simulink model "ASM_Traffic_MultiCore"  (R2026a)
settings: Solver=ode1  StartTime=SIM.tstart.v  StopTime=SIM.tend.v  FixedStep=SIM.StepSize.v
PostLoadFcn:
  | if any(exist('dsrtsu_mdlpostloadfcn', 'file') ~= 0), dsrtsu_mdlpostloadfcn('Execute', bdroot); end
  | try, asm_mdl_postloadfcn(bdroot, 'UpdateModel', 3600); catch, disp(lasterr); end,
InitFcn:
  | , if any(exist('rtifpga_mdlclblib', 'file') ~= 0), rtifpga_mdlclblib('Init', bdroot); end,
  | , if any(exist('dsmpb_private', 'file') ~= 0), dsmpb_private('dsmpb_mdlclblib', 'Init', bdroot); end,
model workspace (MAT data in the model file):
  asmReferencePath = [0 0.01 0.02 0.03 0.04 0.05 0.06 0.07 0.08 0.09 0.1 0.11 ... (350007 elements, 50001x7)]
  roadBounds : Simulink.Parameter (value not decoded)
  safetyAxes : Simulink.Parameter (value not decoded)
undefined symbols (not defined in the file): _to_, a0b2, ASM_BrakeHydraulics_DemoSystems, ASM_VehicleDynamics_DemoSystems, b98103fe8ad365046cd0, BrakeCircuit, controllerConfig, CPT, Crankshaft, DiscIntNeverNeededParam, dsmsi, FinalDriveAssembly, MDL, ModeSignals, mu, Pos_BrakePedal_Maneuver, rad, RefSignals, roadFamilyData, roadFamilyId, s_to_rpm, SIM, SoftECU, Suspension, Tire, Transmission
libraries: ASM_Traffic_lib x135, simulink x98, ASM_Utils_lib x77, ASM_VehicleDynamics_lib x70, ASM_Environment_lib x22, dsmpblib x20, dsmsilib x15, MDLD_Utils_lib x10, ASM_BrakeHydraulics_lib x3, sl_discontinuities x2
(part 33 of 65)

== system ASM_Traffic_MultiCore/VehicleDynamics/Plant/VehicleDynamics/Tire ==
  UnitVec_y_Wheel_CoorSys_V[FL,FR,RL,RR][x;y;z] : Inport
  RotationMatrix_V_to_E_T[3x3] : Inport  Port=2
  Pos_Wheels_CoorSys_E[FL,FR,RL,RR][x,y,z][m] : Inport  Port=3
  v_Abs_WheelBody_CoorSys_V[FL,FR,RL,RR][x;y;z][m|s] : Inport  Port=4
  w_Abs_Wheel_CoorSys_V[FL,FR,RL,RR][x,y,z][rad|s] : Inport  Port=5
  Sw_Tire_Parameter_Set[FL,FR,RL,RR][1|2|3|4] : Inport  Port=6
  Coef_Fric_Road[FL,FR,RL,RR][] : Inport  Port=7
  " Pos_z_CP_CoorSys_E[FL,FR,RL,RR][m]" : Inport  Port=8
  UnitVec_z_CP_CoorSys_E[FL,FR,RL,RR][x;y;z] : Inport  Port=9
  Reset[] : Inport  Port=10
  omega_Wheel[FL,FR,RL,RR][rad|s] : Inport  Port=11
  Sw_r_Tire[1:intern;2:extern] : Inport  Port=12
  r_Tire_extern[m] : Inport  Port=13
  ASMSignalCollector : Subsystem
  Bus Creator1 : BusCreator  Inputs=2
  Demux : Demux  Outputs=[1 1]
  Goto Tag Visibility : GotoTagVisibility  GotoTag=ASMBUS_VehicleDynamics_Tire_FL_ContactPoint
  Goto Tag Visibility1 : GotoTagVisibility  GotoTag=ASMBUS_VehicleDynamics_Tire_FL_Tire
  Goto Tag Visibility10 : GotoTagVisibility  GotoTag=ASMBUS_VehicleDynamics_Tire_RR_ForcesAndTorques
  Goto Tag Visibility16 : GotoTagVisibility  GotoTag=ASMBUS_VehicleDynamics_Tire_FR_ForcesAndTorques
  Goto Tag Visibility2 : GotoTagVisibility  GotoTag=ASMBUS_VehicleDynamics_Tire_FR_ContactPoint
  Goto Tag Visibility3 : GotoTagVisibility  GotoTag=ASMBUS_VehicleDynamics_Tire_FL_ForcesAndTorques
  Goto Tag Visibility4 : GotoTagVisibility  GotoTag=ASMBUS_VehicleDynamics_Tire_RL_ContactPoint
  Goto Tag Visibility5 : GotoTagVisibility  GotoTag=ASMBUS_VehicleDynamics_Tire_RL_Tire
  Goto Tag Visibility6 : GotoTagVisibility  GotoTag=ASMBUS_VehicleDynamics_Tire_FR_Tire
  Goto Tag Visibility7 : GotoTagVisibility  GotoTag=ASMBUS_VehicleDynamics_Tire_RL_ForcesAndTorques
  Goto Tag Visibility8 : GotoTagVisibility  GotoTag=ASMBUS_VehicleDynamics_Tire_RR_ContactPoint
  Goto Tag Visibility9 : GotoTagVisibility  GotoTag=ASMBUS_VehicleDynamics_Tire_RR_Tire
  Mux{1,3..5} (4 alike) : Mux
  Sat_TireParSet : Saturate  UpperLimit=4  LowerLimit=1
  Selector{1..2,14,32} (4 alike) : Selector  InputPortWidth=4  IndexOptions=Index vector (dialog)  Indices=[2]  OutputSizes=1
  Selector{3,9..10,31} (4 alike) : Selector  InputPortWidth=4  IndexOptions=Index vector (dialog)  Indices=[1]  OutputSizes=1
  Selector{7..8,11..13} (5 alike) : Selector  InputPortWidth=12  IndexOptions=Index vector (dialog)  Indices=[4 5 6]  OutputSizes=1
  Selector{15..16,22,33} (4 alike) : Selector  InputPortWidth=4  IndexOptions=Index vector (dialog)  Indices=[3]  OutputSizes=1
  Selector{17..21} (5 alike) : Selector  InputPortWidth=12  IndexOptions=Index vector (dialog)  Indices=[7 8 9]  OutputSizes=1
  Selector{23..25,34} (4 alike) : Selector  InputPortWidth=4  IndexOptions=Index vector (dialog)  Indices=[4]  OutputSizes=1
  Selector{26..30} (5 alike) : Selector  InputPortWidth=12  IndexOptions=Index vector (dialog)  Indices=[10 11 12]  OutputSizes=1
  Selector{4..6,37..38} (5 alike) : Selector  InputPortWidth=12  IndexOptions=Index vector (dialog)  Indices=[1 2 3]  OutputSizes=1
  TIRE_MODE : ASM_VehicleDynamics_lib/VehicleDynamics/Tire/Base/TIRE_MODE  Tag=ASM_SUBCOMPONENT  ModeLeft=MDL.VehicleDynamics.Tire.ModeLeft  ModeRight=MDL.VehicleDynamics.Tire.ModeRight  ASMProperties=struct('Name','TIRE_MODE','Version','1.0','Library','ASM_VehicleDynamics_lib')  ASMInstanceName=tire_mode  ASMInstanceID=1
  Tire_FL : Subsystem
  Tire_FR : Subsystem
  Tire_RL : Subsystem
  Tire_RR : Subsystem
  p[Pa] : Constant  Value=220000
  ASMSignalBus : Outport  VectorParamsAs1DForOutWhenUnconnected=off
  F_Tire_CoorSys_V[FL,FR,RL,RR][x;y;z][N] : Outport  Port=2  VectorParamsAs1DForOutWhenUnconnected=off
  Trq_Tire_CoorSys_V[FL,FR,RL,RR][x;y;z][Nm] : Outport  Port=3  VectorParamsAs1DForOutWhenUnconnected=off
  Stiffness_z_Tire[FL,FR,RL,RR][N|m] : Outport  Port=4  VectorParamsAs1DForOutWhenUnconnected=off
  Trq_Tire_Wheel[FL,FR,RL,RR][Nm] : Outport  Port=5  VectorParamsAs1DForOutWhenUnconnected=off
  wires:
  ASMSignalCollector/1(ASMSignalBus) -> ASMSignalBus/1
  Mux4/1 -> F_Tire_CoorSys_V[FL,FR,RL,RR][x;y;z][N]/1
  Mux1/1 -> Trq_Tire_CoorSys_V[FL,FR,RL,RR][x;y;z][Nm]/1
  Selector10/1 -> Tire_FL/9(omega_Wheel[rad|s])
  omega_Wheel[FL,FR,RL,RR][rad|s]/1 -> Selector24/1, Selector22/1, Selector1/1, Selector10/1
  Selector37/1 -> Tire_FL/8(UnitVec_y_Wheel_CoorSys_V[x;y;z])
  UnitVec_y_Wheel_CoorSys_V[FL,FR,RL,RR][x;y;z]/1 -> Selector30/1, Selector21/1, Selector7/1, Selector37/1
  RotationMatrix_V_to_E_T[3x3]/1 -> Tire_RR/7(RotationMatrix_V_to_E_T[3x3]), Tire_RL/7(RotationMatrix_V_to_E_T[3x3]), Tire_FR/7(RotationMatrix_V_to_E_T[3x3]), Tire_FL/7(RotationMatrix_V_to_E_T[3x3])
  UnitVec_z_CP_CoorSys_E[FL,FR,RL,RR][x;y;z]/1 -> Selector26/1, Selector17/1, Selector11/1, Selector4/1
  " Pos_z_CP_CoorSys_E[FL,FR,RL,RR][m]"/1 -> Selector25/1, Selector16/1, Selector2/1, Selector3/1
  Selector3/1 -> Tire_FL/2(" Pos_z_CP_CoorSys_E[m]")
  Selector9/1 -> Tire_FL/1(Coeff_Fric_Road[])
  Coef_Fric_Road[FL,FR,RL,RR][]/1 -> Selector23/1, Selector15/1, Selector14/1, Selector9/1
  Selector4/1 -> Tire_FL/3(UnitVec_z_CP_CoorSys_E[x;y;z])
  Pos_Wheels_CoorSys_E[FL,FR,RL,RR][x,y,z][m]/1 -> Selector27/1, Selector18/1, Selector12/1, Selector5/1
  Selector5/1 -> Tire_FL/4(Pos_Wheels_CoorSys_E[x;y;z][m])
  v_Abs_WheelBody_CoorSys_V[FL,FR,RL,RR][x;y;z][m|s]/1 -> Selector28/1, Selector19/1, Selector8/1, Selector6/1
  Selector6/1 -> Tire_FL/5(v_Abs_WheelBody_CoorSys_V[x;y;z][m|s])
  w_Abs_Wheel_CoorSys_V[FL,FR,RL,RR][x,y,z][rad|s]/1 -> Selector29/1, Selector20/1, Selector13/1, Selector38/1
  Selector38/1 -> Tire_FL/6(w_Abs_Wheel_CoorSys_V[x;y;z][rad|s])
  Selector14/1 -> Tire_FR/1(Coeff_Fric_Road[])
  Selector2/1 -> Tire_FR/2(" Pos_z_CP_CoorSys_E[m]")
  Selector11/1 -> Tire_FR/3(UnitVec_z_CP_CoorSys_E[x;y;z])
  Selector12/1 -> Tire_FR/4(Pos_Wheels_CoorSys_E[x;y;z][m])
  Selector8/1 -> Tire_FR/5(v_Abs_WheelBody_CoorSys_V[x;y;z][m|s])
  Selector13/1 -> Tire_FR/6(w_Abs_Wheel_CoorSys_V[x;y;z][rad|s])
  Selector7/1 -> Tire_FR/8(UnitVec_y_Wheel_CoorSys_V[x;y;z])
  Selector1/1 -> Tire_FR/9(omega_Wheel[rad|s])
  Selector15/1 -> Tire_RL/1(Coeff_Fric_Road[])
  Selector16/1 -> Tire_RL/2(" Pos_z_CP_CoorSys_E[m]")
  Selector17/1 -> Tire_RL/3(UnitVec_z_CP_CoorSys_E[x;y;z])
  Selector18/1 -> Tire_RL/4(Pos_Wheels_CoorSys_E[x;y;z][m])
  Selector19/1 -> Tire_RL/5(v_Abs_WheelBody_CoorSys_V[x;y;z][m|s])
  Selector20/1 -> Tire_RL/6(w_Abs_Wheel_CoorSys_V[x;y;z][rad|s])
  Selector21/1 -> Tire_RL/8(UnitVec_y_Wheel_CoorSys_V[x;y;z])
  Selector22/1 -> Tire_RL/9(omega_Wheel[rad|s])
  Tire_FL/1(F_Tire[x;y;z][N]) -> Mux4/1
  Tire_FR/1(F_Tire[x;y;z][N]) -> Mux4/2
  Tire_RL/1(F_Tire[x;y;z][N]) -> Mux4/3
  Tire_RR/1(F_Tire[x;y;z][N]) -> Mux4/4
  Tire_FL/2(Trq_Tire[x;y;z][Nm]) -> Mux1/1
  Tire_FR/2(Trq_Tire[x;y;z][Nm]) -> Mux1/2
  Tire_RL/2(Trq_Tire[x;y;z][Nm]) -> Mux1/3
  Tire_RR/2(Trq_Tire[x;y;z][Nm]) -> Mux1/4
  Mux3/1 -> Trq_Tire_Wheel[FL,FR,RL,RR][Nm]/1
  Tire_FL/3(Trq_Tire_Wheel[Nm]) -> Mux3/1
  Tire_FR/3(Trq_Tire_Wheel[Nm]) -> Mux3/2
  Tire_RL/3(Trq_Tire_Wheel[Nm]) -> Mux3/3
  Tire_RR/3(Trq_Tire_Wheel[Nm]) -> Mux3/4
  Sw_Tire_Parameter_Set[FL,FR,RL,RR][1|2|3|4]/1 -> Sat_TireParSet/1
  Selector31/1 -> Tire_FL/10(Sw_Tire_Parameter_Set[1|2|3|4])
  Selector32/1 -> Tire_FR/10(Sw_Tire_Parameter_Set[1|2|3|4])
  Selector33/1 -> Tire_RL/10(Sw_Tire_Parameter_Set[1|2|3|4])
  Selector34/1 -> Tire_RR/10(Sw_Tire_Parameter_Set[1|2|3|4])
  Selector30/1 -> Tire_RR/8(UnitVec_y_Wheel_CoorSys_V[x;y;z])
  Selector24/1 -> Tire_RR/9(omega_Wheel[rad|s])
  Selector29/1 -> Tire_RR/6(w_Abs_Wheel_CoorSys_V[x;y;z][rad|s])
  Selector28/1 -> Tire_RR/5(v_Abs_WheelBody_CoorSys_V[x;y;z][m|s])
  Selector27/1 -> Tire_RR/4(Pos_Wheels_CoorSys_E[x;y;z][m])
  Selector26/1 -> Tire_RR/3(UnitVec_z_CP_CoorSys_E[x;y;z])
  Selector25/1 -> Tire_RR/2(" Pos_z_CP_CoorSys_E[m]")
  Selector23/1 -> Tire_RR/1(Coeff_Fric_Road[])
  Tire_FL/4(Stiffness_z_Tire[N|m]) -> Mux5/1
  Tire_FR/4(Stiffness_z_Tire[N|m]) -> Mux5/2
  Tire_RL/4(Stiffness_z_Tire[N|m]) -> Mux5/3
  Tire_RR/4(Stiffness_z_Tire[N|m]) -> Mux5/4
  Mux5/1 -> Stiffness_z_Tire[FL,FR,RL,RR][N|m]/1
  Reset[]/1 -> Tire_RR/11(Reset[]), Tire_RL/11(Reset[]), Tire_FR/11(Reset[]), Tire_FL/11(Reset[])
  Sat_TireParSet/1 -> Selector34/1, Selector33/1, Selector32/1, Selector31/1
  Demux/1 -> Tire_RL/12(Mode[1Normal|2Mirror|3Symmetric]), Tire_FL/12(Mode[1Normal|2Mirror|3Symmetric])
  p[Pa]/1 -> Tire_RR/13(p[Pa]), Tire_RL/13(p[Pa]), Tire_FR/13(p[Pa]), Tire_FL/13(p[Pa])
  Demux/2 -> Tire_RR/12(Mode[1Normal|2Mirror|3Symmetric]), Tire_FR/12(Mode[1Normal|2Mirror|3Symmetric])
  TIRE_MODE/1 -> Demux/1
  Sw_r_Tire[1:intern;2:extern]/1 -> Bus Creator1/1
  r_Tire_extern[m]/1 -> Bus Creator1/2
  Bus Creator1/1 -> Tire_RR/14(Tire_Switches), Tire_RL/14(Tire_Switches), Tire_FR/14(Tire_Switches), Tire_FL/14(Tire_Switches)

== system ASM_Traffic_MultiCore/VehicleDynamics/Plant/VehicleDynamics/TireMapping_CP ==
  Sw_Tire_Parameter_Set_CP[:][1|2|3|4] : Inport
  Fric_Coeff_CP[:][] : Inport  Port=2
  Pos_z_CP[:][m] : Inport  Port=3
  UnitVec_z_CP[:][x;y;z] : Inport  Port=4
  Selector : Selector  IndexOptions=Index vector (dialog)  Indices=[1:4]  OutputSizes=1
  Selector1 : Selector  IndexOptions=Index vector (dialog)  Indices=[1:4]  OutputSizes=1
  Selector2 : Selector  IndexOptions=Index vector (dialog)  Indices=[1:4]  OutputSizes=1
  Selector3 : Selector  IndexOptions=Index vector (dialog)  Indices=[1:12]  OutputSizes=1
  Sw_Tire_Parameter_Set_CP_Veh[FL;FR;RL;RR][1|2|3|4] : Outport  VectorParamsAs1DForOutWhenUnconnected=off
  Fric_Coeff_CP_Veh[FL;FR;RL;RR][] : Outport  Port=2  VectorParamsAs1DForOutWhenUnconnected=off
  Pos_z_CP_Veh[FL;FR;RL;RR][m] : Outport  Port=3  VectorParamsAs1DForOutWhenUnconnected=off
  UnitVec_z_CP_Veh[FL;FR;RL;RR][x;y;z] : Outport  Port=4  VectorParamsAs1DForOutWhenUnconnected=off
  wires:
  Selector2/1 -> Sw_Tire_Parameter_Set_CP_Veh[FL;FR;RL;RR][1|2|3|4]/1
  Selector3/1 -> UnitVec_z_CP_Veh[FL;FR;RL;RR][x;y;z]/1
  Selector1/1 -> Fric_Coeff_CP_Veh[FL;FR;RL;RR][]/1
  Selector/1 -> Pos_z_CP_Veh[FL;FR;RL;RR][m]/1
  Pos_z_CP[:][m]/1 -> Selector/1
  Fric_Coeff_CP[:][]/1 -> Selector1/1
  UnitVec_z_CP[:][x;y;z]/1 -> Selector3/1
  Sw_Tire_Parameter_Set_CP[:][1|2|3|4]/1 -> Selector2/1

== system ASM_Traffic_MultiCore/VehicleDynamics/Plant/VehicleDynamics/VehicleInits ==
  q_dt_Vehicle_Init[6x1] : Inport
  q_dt_Wheel_Init[:] : Inport  Port=2
  q_Wheel_Init_In[:] : Inport  Port=3
  Bus Selector : BusSelector  OutputSignals=Tire_allSignals.Tire_FL.Tire.r_Dyn_Tire[m],Tire_allSignals.Tire_FR.Tire.r_Dyn_Tire[m],Tire_allSignals.Tire_RL.Tire.r_Dyn_Tire[m],Tire_allSignals.Tire_RR.Tire.r_Dyn_Tire[m]
  Mux : Mux  Inputs=2
  Mux1 : Mux
  Product : Product  Inputs=/*  RndMeth=Zero
  Saturation : Saturate  UpperLimit=inf  LowerLimit=0.01
  Unit Delay : UnitDelay  SampleTime=-1
  v_x_Init[m|s] : Selector  InputPortWidth=6  IndexOptions=Index vector (dialog)  Indices=[1]  OutputSizes=1
  omega_Wheel_Init[:][rad|s] : Outport  VectorParamsAs1DForOutWhenUnconnected=off
  q_dt_Init[:] : Outport  Port=2  VectorParamsAs1DForOutWhenUnconnected=off
  q_Wheel_Init[:] : Outport  Port=3  VectorParamsAs1DForOutWhenUnconnected=off
  wires:
  q_dt_Vehicle_Init[6x1]/1 -> v_x_Init[m|s]/1, Mux/1
  Mux1/1 -> Saturation/1
  Bus Selector/4 -> Mux1/4  "<r_Dyn_Tire[m]>"
  Bus Selector/3 -> Mux1/3  "<r_Dyn_Tire[m]>"
  Bus Selector/2 -> Mux1/2  "<r_Dyn_Tire[m]>"
  v_x_Init[m|s]/1 -> Product/2
  Mux/1 -> q_dt_Init[:]/1
  q_Wheel_Init_In[:]/1 -> q_Wheel_Init[:]/1
  q_dt_Wheel_Init[:]/1 -> Mux/2
  Saturation/1 -> Product/1
  Bus Selector/1 -> Mux1/1  "<r_Dyn_Tire[m]>"
  Unit Delay/1 -> omega_Wheel_Init[:][rad|s]/1
  Product/1 -> Unit Delay/1
  [ASMBUS_VehicleDynamics_Tire] -> Bus Selector/1

== system ASM_Traffic_MultiCore/VehicleDynamics/Plant/VehicleDynamics/VehicleMovement ==
  F_Aero_CoorSys_V[x;y;z][N] : Inport
  Trq_Aero_CoorSys_V[x;y;z][Nm] : Inport  Port=2
  F_Tire_CoorSys_V[FL,FR,RL,RR][x;y;z][N] : Inport  Port=3
  Trq_Tire_CoorSys_V[FL,FR,RL,RR][x;y;z][Nm] : Inport  Port=4
  Stiffness_z_Tire[FL,FR,RL,RR][N|m] : Inport  Port=5
  w_Wheel[FL,FR,RL,RR][x;y;z][rad|s] : Inport  Port=6
  Trq_Shaft_CoorSys_V[FL,FR,RL,RR][x;y;z][Nm] : Inport  Port=7
  gF_Susp[q1_Front;q2_Front;q1_Rear;q2_Rear][] : Inport  Port=8
  Pos_Wheel[FL,FR,RL,RR][x;y;z][m] : Inport  Port=9
  w_Rel_WheelBody[FL,FR,RL,RR][x y z][rad|s] : Inport  Port=10
  v_Rel_WheelBody[FL,FR,RL,RR][x;y;z][m|s] : Inport  Port=11
  Pos_Vehicle_Init_CoorSys_E[x;y;z][m] : Inport  Port=12
  Angle_V_Init_CoorSys_E[x;y;z][rad] : Inport  Port=13
  Reset[] : Inport  Port=14
  KeepVehiclePosition[0|1] : Inport  Port=15
  gRear_dq_Rear_dt[2x2][] : Inport  Port=16
  gFront_dq_Front_dt[2x2][] : Inport  Port=17
  SuspensionKinematicsRelations_Rear : Inport  Port=18
  SuspensionKinematicsRelations_Front : Inport  Port=19
  F_External_CoorSys_V[x,y,z][N] : Inport  Port=20
  Trq_External_CoorSys_V[x,y,z][Nm] : Inport  Port=21
  Stabilization_F_External[3X6] : Inport  Port=22
  Stabilization_Trq_External[3X6] : Inport  Port=23
  q_dt_Init[:] : Inport  Port=24
  q_Wheel_Init[:] : Inport  Port=25
  ASMSignalCollector : Subsystem
  Bus Selector1 : BusSelector  OutputSignals=Pos_RL_Wheel_dq_Rear[q1;q2][x;y;z][],w_Rel_RL_Wheel_dq_Rear_dt[q1;q2][x;y;z][],Pos_RR_Wheel_dq_Rear[q1;q2][x;y;z][],w_Rel_RR_Wheel_dq_Rear[q1;q2][x;y;z][]
  Bus Selector2 : BusSelector  OutputSignals=Pos_FL_Wheel_dq_Front[q1;q2][x;y;z][],w_Rel_FL_Wheel_dq_Front_dt[q1;q2][x;y;z][],Pos_FR_Wheel_dq_Front[q1;q2][x;y;z][],w_Rel_FR_Wheel_dq_Front[q1;q2][x;y;z][]
  COORDINATE_TRANSFORMATION : ASM_VehicleDynamics_lib/VehicleDynamics/VehicleMovement/COORDINATE_TRANSFORMATION  Tag=ASM_SUBCOMPONENT  StepSize=SIM.StepSize  ASMProperties=struct('Name','COORDINATE_TRANSFORMATION','Version','5.0','Library','ASM_VehicleDynamics_lib')  ASMInstanceName=coordinate_transformation  ASMInstanceID=1
  Goto Tag Visibility : GotoTagVisibility  GotoTag=ASMBUS_VehicleDynamics_VehicleMotion
  Goto Tag Visibility1 : GotoTagVisibility  GotoTag=ASMBUS_VehicleDynamics_CoGAndWheelVelocities
  Goto Tag Visibility2 : GotoTagVisibility  GotoTag=ASMBUS_VehicleDynamics_SensorMotion
  Goto Tag Visibility3 : GotoTagVisibility  GotoTag=ASMBUS_VehicleDynamics_MassForcesAndTorques
  Goto Tag Visibility4 : GotoTagVisibility  GotoTag=ASMBUS_VehicleDynamics_CoordinateTransformation
  Goto Tag Visibility5 : GotoTagVisibility  GotoTag=ASMBUS_VehicleDynamics_VehicleMass
  J : Constant  Value=zeros(3,3)
  MASS_FORCES_AND_TORQUES : ASM_VehicleDynamics_lib/VehicleDynamics/VehicleMovement/MASS_FORCES_AND_TORQUES  Tag=ASM_SUBCOMPONENT  ASMProperties=struct('Name','MASS_FORCES_AND_TORQUES','Version','3.0','Library','ASM_VehicleDynamics_lib')  ASMInstanceName=mass_forces_and_torques  ASMInstanceID=1
  OR : Subsystem
  SENSOR_MOTION : ASM_VehicleDynamics_lib/VehicleDynamics/VehicleMovement/SENSOR_MOTION  Tag=ASM_SUBCOMPONENT  Const_PosVec_Sensor1=MDL.VehicleDynamics.VehicleMovement.SensorMotion.Const_PosVec_Sensor1  Const_PosVec_Sensor2=MDL.VehicleDynamics.VehicleMovement.SensorMotion.Const_PosVec_Sensor2  Const_PosVec_Sensor3=MDL.VehicleDynamics.VehicleMovement.SensorMotion.Const_PosVec_Sensor3  Const_PosVec_Sensor4=MDL.VehicleDynamics.VehicleMovement.SensorMotion.Const_PosVec_Sensor4  ASMProperties=struct('Name','SENSOR_MOTION','Version','5.0','Library','ASM_VehicleDynamics_lib')  ASMInstanceName=sensor_motion  ASMInstanceID=1
  Selector1 : Selector  InputPortWidth=15  IndexOptions=Index vector (dialog)  Indices=[4:15]  OutputSizes=1
  Selector2 : Selector  InputPortWidth=15  IndexOptions=Index vector (dialog)  Indices=[4:15]  OutputSizes=1
  Selector3 : Selector  InputPortWidth=15  IndexOptions=Index vector (dialog)  Indices=[4:15]  OutputSizes=1
  Sw_TestBenchMode[1Vehicle|2TestBench] : Constant
  Terminator : Terminator
  VEHICLE_AND_WHEEL_VELOCITIES : ASM_VehicleDynamics_lib/VehicleDynamics/VehicleMovement/VEHICLE_AND_WHEEL_VELOCITIES  Tag=ASM_SUBCOMPONENT  ASMProperties=struct('Name','VEHICLE_AND_WHEEL_VELOCITIES','Version','1.0','Library','ASM_VehicleDynamics_lib')  ASMInstanceName=vehicle_and_wheel_velocities  ASMInstanceID=1
  VEHICLE_MASS_AND_ADDITIONAL_LOADS : ASM_VehicleDynamics_lib/VehicleDynamics/VehicleMovement/VEHICLE_MASS_AND_ADDITIONAL_LOADS  Tag=ASM_SUBCOMPONENT  Const_m_Vehicle=MDL.VehicleDynamics.Vehicle.Const_m_Vehicle  Const_PosVec_CoG_Vehicle=MDL.VehicleDynamics.Vehicle.Const_PosVec_CoG_Vehicle  Const_Inertia_Tensor_Vehicle=MDL.VehicleDynamics.Vehicle.Const_Inertia_Tensor_Vehicle  Const_m_AddLoad1=MDL.VehicleDynamics.VehicleMovement.AddLoad1.Const_m_AddLoad1  Const_PosVec_CoG_AddLoad1=MDL.VehicleDynamics.VehicleMovement.AddLoad1.Const_PosVec_CoG_AddLoad1  Const_Inertia_Tensor_AddLoad1=MDL.VehicleDynamics.VehicleMovement.AddLoad1.Const_Inertia_Tensor_AddLoad1  Sw_AddLoad1=MDL.VehicleDynamics.VehicleMovement.AddLoad1.Sw_AddLoad1  Const_m_AddLoad2=MDL.VehicleDynamics.VehicleMovement.AddLoad2.Const_m_AddLoad2  Const_PosVec_CoG_AddLoad2=MDL.VehicleDynamics.VehicleMovement.AddLoad2.Const_PosVec_CoG_AddLoad2  Const_Inertia_Tensor_AddLoad2=MDL.VehicleDynamics.VehicleMovement.AddLoad2.Const_Inertia_Tensor_AddLoad2  Sw_AddLoad2=MDL.VehicleDynamics.VehicleMovement.AddLoad2.Sw_AddLoad2  Const_m_AddLoad3=MDL.VehicleDynamics.VehicleMovement.AddLoad3.Const_m_AddLoad3  Const_PosVec_CoG_AddLoad3=MDL.VehicleDynamics.VehicleMovement.AddLoad3.Const_PosVec_CoG_AddLoad3  Const_Inertia_Tensor_AddLoad3=MDL.VehicleDynamics.VehicleMovement.AddLoad3.Const_Inertia_Tensor_AddLoad3  Sw_AddLoad3=MDL.VehicleDynamics.VehicleMovement.AddLoad3.Sw_AddLoad3  Const_m_AddLoad4=MDL.VehicleDynamics.VehicleMovement.AddLoad4.Const_m_AddLoad4  Const_PosVec_CoG_AddLoad4=MDL.VehicleDynamics.VehicleMovement.AddLoad4.Const_PosVec_CoG_AddLoad4  Const_Inertia_Tensor_AddLoad4=MDL.VehicleDynamics.VehicleMovement.AddLoad4.Const_Inertia_Tensor_AddLoad4  Sw_AddLoad4=MDL.VehicleDynamics.VehicleMovement.AddLoad4.Sw_AddLoad4  Const_m_AddLoad5=MDL.VehicleDynamics.VehicleMovement.AddLoad5.Const_m_AddLoad5  Const_PosVec_CoG_AddLoad5=MDL.VehicleDynamics.VehicleMovement.AddLoad5.Const_PosVec_CoG_AddLoad5  Const_Inertia_Tensor_AddLoad5=MDL.VehicleDynamics.VehicleMovement.AddLoad5.Const_Inertia_Tensor_AddLoad5  Sw_AddLoad5=MDL.VehicleDynamics.VehicleMovement.AddLoad5.Sw_AddLoad5  Const_m_AddLoad6=MDL.VehicleDynamics.VehicleMovement.AddLoad6.Const_m_AddLoad6  Const_PosVec_CoG_AddLoad6=MDL.VehicleDynamics.VehicleMovement.AddLoad6.Const_PosVec_CoG_AddLoad6  Const_Inertia_Tensor_AddLoad6=MDL.VehicleDynamics.VehicleMovement.AddLoad6.Const_Inertia_Tensor_AddLoad6  Sw_AddLoad6=MDL.VehicleDynamics.VehicleMovement.AddLoad6.Sw_AddLoad6  ASMProperties=struct('Name','VEHICLE_MASS_AND_ADDITIONAL_LOADS','Version','4.0','Library','ASM_VehicleDynamics_lib')  ASMInstanceName=vehicle_mass_and_additional_loads  ASMInstanceID=1
  VEHICLE_MOTION_CAR : ASM_VehicleDynamics_lib/VehicleDynamics/VehicleMovement/VEHICLE_MOTION_CAR  Tag=ASM_SUBCOMPONENT  StepSize=SIM.StepSize  ASMProperties=struct('Name','VEHICLE_MOTION_CAR','Version','6.0','Library','ASM_VehicleDynamics_lib')  ASMInstanceName=vehicle_motion_car  ASMInstanceID=1
  m : Constant  Value=0
  r_CoG : Constant  Value=[0 0 0]
  ASMSignalBus : Outport  VectorParamsAs1DForOutWhenUnconnected=off
  v_Abs_Vehicle_CoG[x;y;z][m|s] : Outport  Port=2  VectorParamsAs1DForOutWhenUnconnected=off
  RotationMatrix_V_to_E_T[3x3] : Outport  Port=3  VectorParamsAs1DForOutWhenUnconnected=off
  Pos_Wheels_CoorSys_E[FL,FR,RL,RR][x;y;z][m] : Outport  Port=4  VectorParamsAs1DForOutWhenUnconnected=off
  v_Abs_WheelBody_CoorSys_V[FL,FR,RL,RR][x y z][m|s] : Outport  Port=5  VectorParamsAs1DForOutWhenUnconnected=off
  w_Abs_Wheel_CoorSys_V[FL,FR,RL,RR][x,y,z][rad|s] : Outport  Port=6  VectorParamsAs1DForOutWhenUnconnected=off
  F_Gyroscopic[FL,FR,RL,RR][x;y;z][N] : Outport  Port=7  VectorParamsAs1DForOutWhenUnconnected=off
  Trq_Gyroscopic[FL,FR,RL,RR][x;y;z][Nm] : Outport  Port=8  VectorParamsAs1DForOutWhenUnconnected=off
  F_Gravitational[FL,FR,RL,RR][x;y;z][N] : Outport  Port=9  VectorParamsAs1DForOutWhenUnconnected=off
  q_Wheel_dt[q1_Front;q2_Front;q1_Rear;q2_Rear][] : Outport  Port=10  VectorParamsAs1DForOutWhenUnconnected=off
  q_Wheel[q1_Front;q2_Front;q1_Rear;q2_Rear][] : Outport  Port=11  VectorParamsAs1DForOutWhenUnconnected=off
  tag scope: ASMBUS_VehicleDynamics_CoGAndWheelVelocities=scoped, ASMBUS_VehicleDynamics_CoordinateTransformation=scoped, ASMBUS_VehicleDynamics_MassForcesAndTorques=scoped, ASMBUS_VehicleDynamics_SensorMotion=scoped, ASMBUS_VehicleDynamics_VehicleMass=global, ASMBUS_VehicleDynamics_VehicleMotion=scoped
  wires:
  COORDINATE_TRANSFORMATION/1 -> [ASMBUS_VehicleDynamics_CoordinateTransformation]
  VEHICLE_AND_WHEEL_VELOCITIES/1 -> [ASMBUS_VehicleDynamics_CoGAndWheelVelocities]
  VEHICLE_MOTION_CAR/1 -> [ASMBUS_VehicleDynamics_VehicleMotion]
  VEHICLE_AND_WHEEL_VELOCITIES/3 -> w_Abs_Wheel_CoorSys_V[FL,FR,RL,RR][x,y,z][rad|s]/1
  VEHICLE_AND_WHEEL_VELOCITIES/5 -> MASS_FORCES_AND_TORQUES/2, v_Abs_Vehicle_CoG[x;y;z][m|s]/1
  VEHICLE_AND_WHEEL_VELOCITIES/4 -> MASS_FORCES_AND_TORQUES/1, v_Abs_WheelBody_CoorSys_V[FL,FR,RL,RR][x y z][m|s]/1
  VEHICLE_AND_WHEEL_VELOCITIES/6 -> MASS_FORCES_AND_TORQUES/3
  MASS_FORCES_AND_TORQUES/3 -> Selector1/1, VEHICLE_MOTION_CAR/14
  MASS_FORCES_AND_TORQUES/2 -> Selector2/1, VEHICLE_MOTION_CAR/15
  VEHICLE_MOTION_CAR/6 -> VEHICLE_AND_WHEEL_VELOCITIES/2, MASS_FORCES_AND_TORQUES/4, COORDINATE_TRANSFORMATION/4, SENSOR_MOTION/4
  VEHICLE_MOTION_CAR/7 -> COORDINATE_TRANSFORMATION/3, SENSOR_MOTION/3, VEHICLE_AND_WHEEL_VELOCITIES/1
  MASS_FORCES_AND_TORQUES/1 -> [ASMBUS_VehicleDynamics_MassForcesAndTorques]
  VEHICLE_MASS_AND_ADDITIONAL_LOADS/1 -> [ASMBUS_VehicleDynamics_VehicleMass]
  VEHICLE_MASS_AND_ADDITIONAL_LOADS/4 -> VEHICLE_AND_WHEEL_VELOCITIES/7, VEHICLE_MOTION_CAR/10
  VEHICLE_MASS_AND_ADDITIONAL_LOADS/3 -> MASS_FORCES_AND_TORQUES/9, VEHICLE_MOTION_CAR/11
  VEHICLE_MASS_AND_ADDITIONAL_LOADS/2 -> MASS_FORCES_AND_TORQUES/8, VEHICLE_MOTION_CAR/12
  VEHICLE_MOTION_CAR/2 -> q_Wheel_dt[q1_Front;q2_Front;q1_Rear;q2_Rear][]/1
  w_Rel_WheelBody[FL,FR,RL,RR][x y z][rad|s]/1 -> VEHICLE_AND_WHEEL_VELOCITIES/5
  v_Rel_WheelBody[FL,FR,RL,RR][x;y;z][m|s]/1 -> MASS_FORCES_AND_TORQUES/5, VEHICLE_AND_WHEEL_VELOCITIES/4
  w_Wheel[FL,FR,RL,RR][x;y;z][rad|s]/1 -> MASS_FORCES_AND_TORQUES/6, VEHICLE_AND_WHEEL_VELOCITIES/6
  VEHICLE_MOTION_CAR/4 -> SENSOR_MOTION/1
  VEHICLE_MOTION_CAR/5 -> SENSOR_MOTION/2
  SENSOR_MOTION/1 -> [ASMBUS_VehicleDynamics_SensorMotion]
  MASS_FORCES_AND_TORQUES/4 -> Selector3/1, VEHICLE_MOTION_CAR/13
  VEHICLE_AND_WHEEL_VELOCITIES/2 -> Terminator/1
  COORDINATE_TRANSFORMATION/2 -> Pos_Wheels_CoorSys_E[FL,FR,RL,RR][x;y;z][m]/1
  COORDINATE_TRANSFORMATION/3 -> RotationMatrix_V_to_E_T[3x3]/1
  Pos_Vehicle_Init_CoorSys_E[x;y;z][m]/1 -> COORDINATE_TRANSFORMATION/5
  Angle_V_Init_CoorSys_E[x;y;z][rad]/1 -> COORDINATE_TRANSFORMATION/6
  COORDINATE_TRANSFORMATION/4 -> MASS_FORCES_AND_TORQUES/7, SENSOR_MOTION/5
  VEHICLE_MOTION_CAR/3 -> q_Wheel[q1_Front;q2_Front;q1_Rear;q2_Rear][]/1
  Reset[]/1 -> ASMSignalCollector/1(Reset[]), COORDINATE_TRANSFORMATION/1, OR/2(In2)
  gF_Susp[q1_Front;q2_Front;q1_Rear;q2_Rear][]/1 -> VEHICLE_MOTION_CAR/2
  Pos_Wheel[FL,FR,RL,RR][x;y;z][m]/1 -> COORDINATE_TRANSFORMATION/2, VEHICLE_AND_WHEEL_VELOCITIES/3, VEHICLE_MOTION_CAR/3
  F_Tire_CoorSys_V[FL,FR,RL,RR][x;y;z][N]/1 -> VEHICLE_MOTION_CAR/4
  Trq_Tire_CoorSys_V[FL,FR,RL,RR][x;y;z][Nm]/1 -> VEHICLE_MOTION_CAR/5
  F_Aero_CoorSys_V[x;y;z][N]/1 -> VEHICLE_MOTION_CAR/6
  Trq_Aero_CoorSys_V[x;y;z][Nm]/1 -> VEHICLE_MOTION_CAR/7
  Stiffness_z_Tire[FL,FR,RL,RR][N|m]/1 -> VEHICLE_MOTION_CAR/8
  Trq_Shaft_CoorSys_V[FL,FR,RL,RR][x;y;z][Nm]/1 -> VEHICLE_MOTION_CAR/9
  gFront_dq_Front_dt[2x2][]/1 -> VEHICLE_MOTION_CAR/24
  gRear_dq_Rear_dt[2x2][]/1 -> VEHICLE_MOTION_CAR/25
  SuspensionKinematicsRelations_Front/1 -> Bus Selector2/1
  Bus Selector2/1 -> VEHICLE_MOTION_CAR/16  "<Pos_FL_Wheel_dq_Front[q1;q2][x;y;z][]>"
  Bus Selector2/2 -> VEHICLE_MOTION_CAR/17  "<w_Rel_FL_Wheel_dq_Front_dt[q1;q2][x;y;z][]>"
  Bus Selector2/3 -> VEHICLE_MOTION_CAR/18  "<Pos_FR_Wheel_dq_Front[q1;q2][x;y;z][]>"
  Bus Selector2/4 -> VEHICLE_MOTION_CAR/19  "<w_Rel_FR_Wheel_dq_Front[q1;q2][x;y;z][]>"
  Bus Selector1/1 -> VEHICLE_MOTION_CAR/20  "<Pos_RL_Wheel_dq_Rear[q1;q2][x;y;z][]>"
  Bus Selector1/2 -> VEHICLE_MOTION_CAR/21  "<w_Rel_RL_Wheel_dq_Rear_dt[q1;q2][x;y;z][]>"
  Bus Selector1/3 -> VEHICLE_MOTION_CAR/22  "<Pos_RR_Wheel_dq_Rear[q1;q2][x;y;z][]>"
  Bus Selector1/4 -> VEHICLE_MOTION_CAR/23  "<w_Rel_RR_Wheel_dq_Rear[q1;q2][x;y;z][]>"
  SuspensionKinematicsRelations_Rear/1 -> Bus Selector1/1
  ASMSignalCollector/1(ASMSignalBus) -> ASMSignalBus/1
  Selector2/1 -> Trq_Gyroscopic[FL,FR,RL,RR][x;y;z][Nm]/1
  Selector1/1 -> F_Gyroscopic[FL,FR,RL,RR][x;y;z][N]/1
  Selector3/1 -> F_Gravitational[FL,FR,RL,RR][x;y;z][N]/1
  F_External_CoorSys_V[x,y,z][N]/1 -> VEHICLE_MOTION_CAR/26
  Trq_External_CoorSys_V[x,y,z][Nm]/1 -> VEHICLE_MOTION_CAR/27
  Stabilization_F_External[3X6]/1 -> VEHICLE_MOTION_CAR/28
  Stabilization_Trq_External[3X6]/1 -> VEHICLE_MOTION_CAR/29
  Sw_TestBenchMode[1Vehicle|2TestBench]/1 -> VEHICLE_MOTION_CAR/30
  KeepVehiclePosition[0|1]/1 -> OR/1(In1)
  OR/1(Out) -> VEHICLE_MOTION_CAR/1
  q_dt_Init[:]/1 -> VEHICLE_MOTION_CAR/31
  q_Wheel_Init[:]/1 -> VEHICLE_MOTION_CAR/32
  COORDINATE_TRANSFORMATION/5 -> SENSOR_MOTION/6
  J/1 -> VEHICLE_MASS_AND_ADDITIONAL_LOADS/3
  r_CoG/1 -> VEHICLE_MASS_AND_ADDITIONAL_LOADS/2
  m/1 -> VEHICLE_MASS_AND_ADDITIONAL_LOADS/1

== system ASM_Traffic_MultiCore/VehicleDynamics/Plant/VehicleDynamics/avoid_incomplete_trace2source ==
  In1 : Inport
  DummyGain : Gain
  Out1 : Outport
  wires:
  DummyGain/1 -> Out1/1
  In1/1 -> DummyGain/1

== system ASM_Traffic_MultiCore/VehicleDynamics/Plant/VehicleDynamics/avoid_incomplete_trace2source1 ==
  In1 : Inport
  DummyGain : Gain
  Out1 : Outport
  wires:
  DummyGain/1 -> Out1/1
  In1/1 -> DummyGain/1

== system ASM_Traffic_MultiCore/VehicleDynamics/Plant/VehicleDynamics/avoid_incomplete_trace2source2 ==
  In1 : Inport
  DummyGain : Gain
  Out1 : Outport
  wires:
  DummyGain/1 -> Out1/1
  In1/1 -> DummyGain/1
